simulink model "ex_04_2_sim"  (R2024b)
settings: Solver=VariableStepAuto  StartTime=0.0  StopTime=10.0  RelTol=1e-3
undefined symbols (not defined in the file or in its folder): A_d, A_v, B_d, B_v, C_d, C_v, D_d, d_start, D_v, gain1, gain2, gain6, gain7, k_x1, k_x2, kyita1, kyita2, kyita3, r, v_start
settings Model: Creator=54238  LastModifiedBy=54238

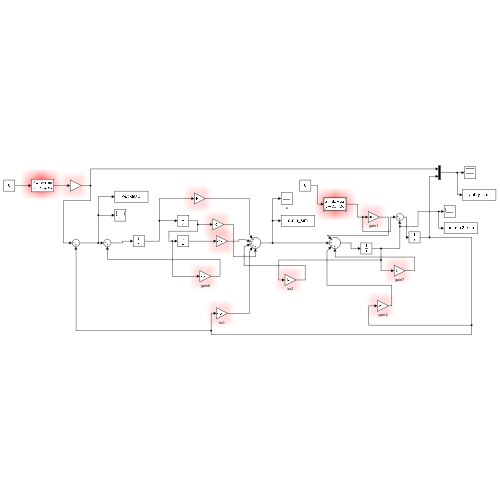
[thumbnail: Simulink's stored preview of the top-level diagram]
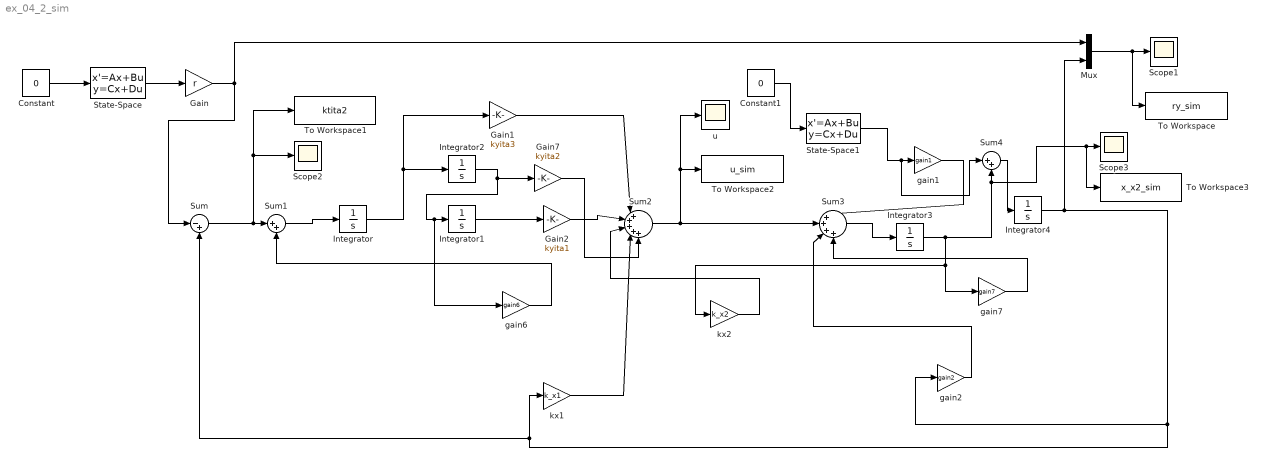
== system ex_04_2_sim ==
  Constant : Constant  Value=0
  Constant1 : Constant  Value=0
  Gain : Gain  Gain=r
  Gain1 : Gain  Gain=kyita3
  Gain2 : Gain  Gain=kyita1
  Gain7 : Gain  Gain=kyita2
  Integrator{,1..4} (5 alike) : Integrator
  Mux : Mux  Inputs=2
  Scope1 : Scope
  Scope2 : Scope
  Scope3 : Scope
  State-Space : StateSpace  A=A_v  B=B_v  C=C_v  D=D_v  InitialCondition=v_start
  State-Space1 : StateSpace  A=A_d  B=B_d  C=C_d  D=D_d  InitialCondition=d_start
  Sum : Sum  Inputs=|-+
  Sum1 : Sum  Inputs=|++
  Sum2 : Sum  Inputs=|+++++
  Sum3 : Sum  Inputs=|++++
  Sum4 : Sum  Inputs=|++
  To Workspace : ToWorkspace  VariableName=ry_sim  SaveFormat=Timeseries  SampleTime=-1
  To Workspace1 : ToWorkspace  VariableName=ktita2  SaveFormat=Timeseries  SampleTime=-1
  To Workspace2 : ToWorkspace  VariableName=u_sim  SaveFormat=Timeseries  SampleTime=-1
  To Workspace3 : ToWorkspace  VariableName=x_x2_sim  SaveFormat=Timeseries  SampleTime=-1
  gain1 : Gain  Gain=gain1
  gain2 : Gain  Gain=gain2
  gain6 : Gain  Gain=gain6
  gain7 : Gain  Gain=gain7
  kx1 : Gain  Gain=k_x1
  kx2 : Gain  Gain=k_x2
  u : Scope
  wires:
  Gain1/1 -> Sum2/1
  Integrator4/1 -> gain2/1, kx1/1, Sum/2, Mux/2
  Gain2/1 -> Sum2/2
  Sum2/1 -> Sum3/2, u/1, To Workspace2/1
  Sum1/1 -> Integrator/1
  Integrator1/1 -> Gain2/1
  State-Space/1 -> Gain/1
  Integrator/1 -> Integrator2/1, Gain1/1
  Gain/1 -> Mux/1, Sum/1
  Sum/1 -> To Workspace1/1, Scope2/1, Sum1/1
  gain6/1 -> Sum1/2
  Mux/1 -> To Workspace/1, Scope1/1
  kx1/1 -> Sum2/4
  Integrator2/1 -> gain6/1, Integrator1/1, Gain7/1
  Gain7/1 -> Sum2/5
  Sum3/1 -> Integrator3/1
  State-Space1/1 -> Sum4/1, gain1/1
  gain1/1 -> Sum3/1
  Sum4/1 -> Integrator4/1
  kx2/1 -> Sum2/3
  Integrator3/1 -> To Workspace3/1, Scope3/1, Sum4/2, gain7/1, kx2/1
  gain7/1 -> Sum3/4
  gain2/1 -> Sum3/3
  Constant/1 -> State-Space/1
  Constant1/1 -> State-Space1/1
